simulink model "buck_boost_conversor"  (R2024b)
settings: Solver=ode23tb  StartTime=0.0  StopTime=0.05  MaxStep=500e-9  RelTol=1e-3
values from neighbouring files (symbols this model uses):
  Ap = Am    [buck_boost_parametros.m]
  Bp = [Bm (A1-A2)*Xbb+(B1-B2)*U]    [buck_boost_parametros.m]
  Cp = Cm    [buck_boost_parametros.m]
  Ep = [Em (C1-C2)*Xbb+(E1-E2)*U]    [buck_boost_parametros.m]
libraries: spsSeriesRLCBranchLib x3, spsCurrentMeasurementLib x1, spsDiodeLib x1, spsIGBTLib x1, spsControlledVoltageSourceLib x1, spsVoltageMeasurementLib x1, sps_lib x1
settings Model: Creator=leona  LastModifiedBy=Seu Computador

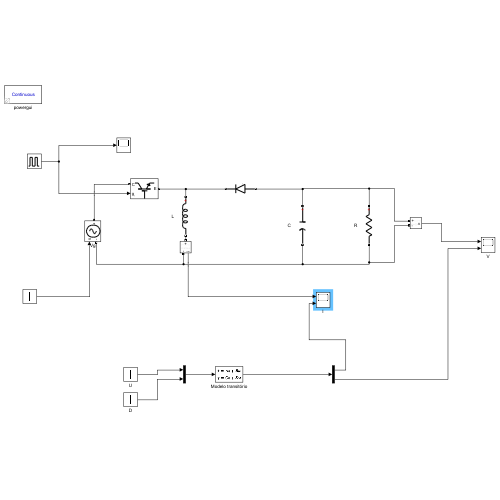
[thumbnail: Simulink's stored preview of the top-level diagram]
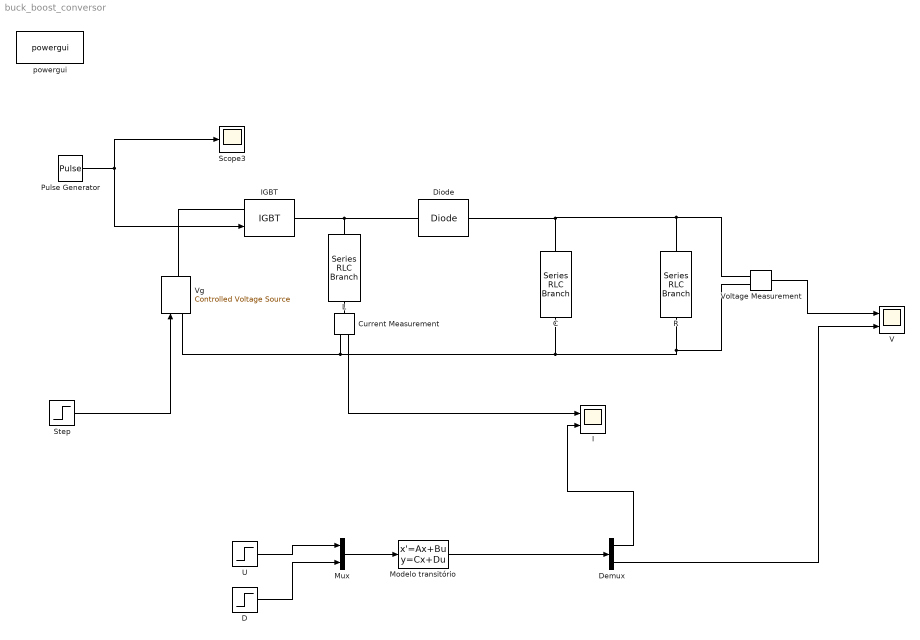
== system buck_boost_conversor ==
  C : spsSeriesRLCBranchLib/Series RLC Branch  LConnTagsString=__new0  RConnTagsString=__new0  BranchType=C  Resistance=1  Inductance=1e-3  SetiL0=off  InitialCurrent=0  Capacitance=100e-6  Setx0=off  InitialVoltage=0  Measurements=None
  Current Measurement : spsCurrentMeasurementLib/Current Measurement  PhasorSimulation=off  OutputType=Complex  PSBequivalent=0
  D : Step  Time=0  After=0.0000005  SampleTime=0
  Demux : Demux  Outputs=2
  Diode : spsDiodeLib/Diode  Ron=1e-9  Lon=0  Vf=0  IC=0  UseSnubber=0  Rs=0  Cs=0  Measurements=off
  I : Scope  NumInputPorts=2
  IGBT : spsIGBTLib/IGBT  Ron=1e-9  Lon=0  Vf=0  Tf=1e-6  Tt=2e-6  IC=0  Rs=0  Cs=0  Measurements=off
  L : spsSeriesRLCBranchLib/Series RLC Branch  LConnTagsString=__new0  RConnTagsString=__new0  BranchType=L  Resistance=1e-10  Inductance=1059e-6  SetiL0=off  InitialCurrent=0  Capacitance=0  Setx0=off  InitialVoltage=0  Measurements=None
  Modelo transitório : StateSpace  A=Ap  B=Bp  C=Cp  D=Ep  InitialCondition=0  AllowTunableDMatrix=on
  Mux : Mux  Inputs=2
  Pulse Generator : DiscretePulseGenerator  PulseType=Time based  Period=1/20000  PulseWidth=40
  R : spsSeriesRLCBranchLib/Series RLC Branch  LConnTagsString=__new0  RConnTagsString=__new0  BranchType=R  Resistance=10  Inductance=1e-3  SetiL0=off  InitialCurrent=0  Capacitance=1e-6  Setx0=off  InitialVoltage=0  Measurements=None
  Scope3 : Scope
  Step : Step  Time=0  After=100  SampleTime=0
  U : Step  Time=0  After=100  SampleTime=0
  V : Scope  NumInputPorts=2
  Vg : spsControlledVoltageSourceLib/Controlled Voltage Source  Initialize=on  Source_Type=DC  Amplitude=0  Phase=0  Frequency=0  Measurements=None
  Voltage Measurement : spsVoltageMeasurementLib/Voltage Measurement  PhasorSimulation=off  OutputType=Complex  PSBequivalent=0
  powergui : sps_lib/powergui  Priority=1  SimulationMode=Continuous  SampleTime=50e-6  frequency=60  Iterations=50  frequencyindice=0  Pbase=100e6  ErrMax=1e-4  UnitsV=kV  UnitsW=MW  buscounter=0  FunctionMessages=off  echomessages=off  EnableUseOfTLC=off  CurrentSourceSwitches=off  DisableSnubberDevices=off  DisableRonSwitches=off  DisableVfSwitches=off  DisplayEquations=off  AutomaticDiscreteSolvers=off  SolverType=Tustin/Backward Euler (TBE)  Interpol=off  ExternalGateDelay=off  methode=off  Ts=100  x0status=blocks  SPID=on  SwTol=0  HookPort=off  NonlinearTolerance=1e-4  nMaxIteration=100  ContinueOnMaxIteration=off  RestoreLinks=warning  ResistiveCurrentMeasurement=off  Frange=[0:2:500]  Ylog=off  Xlog=on  ShowGrid=off  save=off  variable=ZData  structure=0  ZoomFFT=off  StartTime=0.0  cycles=1  DisplayStyle=1  fundamental=60  FreqAxis=off  MaxFrequency=1000  frequencyindicesteady=1  RmsSteady=1  display=off
  wires:
  Step/1 -> Vg/1
  Pulse Generator/1 -> Scope3/1, IGBT/1
  Current Measurement/1 -> I/1
  Voltage Measurement/1 -> V/1
  Demux/1 -> I/2
  Demux/2 -> V/2
  U/1 -> Mux/1
  D/1 -> Mux/2
  Mux/1 -> Modelo transitório/1
  Modelo transitório/1 -> Demux/1
  connections:
  Vg/LConn1 -- Current Measurement/RConn1 -- C/RConn1 -- Voltage Measurement/LConn2 -- R/RConn1
  C/LConn1 -- Diode/LConn1 -- Voltage Measurement/LConn1 -- R/LConn1
  Diode/RConn1 -- IGBT/RConn1 -- L/LConn1
  Current Measurement/LConn1 -- L/RConn1
  Vg/RConn1 -- IGBT/LConn1
